simulink model "assm1023"  (R2017a)
settings: Solver=VariableStepAuto  StartTime=0.0  StopTime=inf  RelTol=1e-3
libraries: mblibv1 x33, simulink x5
settings Model: Creator=phoenix  LastModifiedBy=phoenix
settings SimMechanicsCC: VisOnUpdateDiagram=on  VisDuringSimulation=on

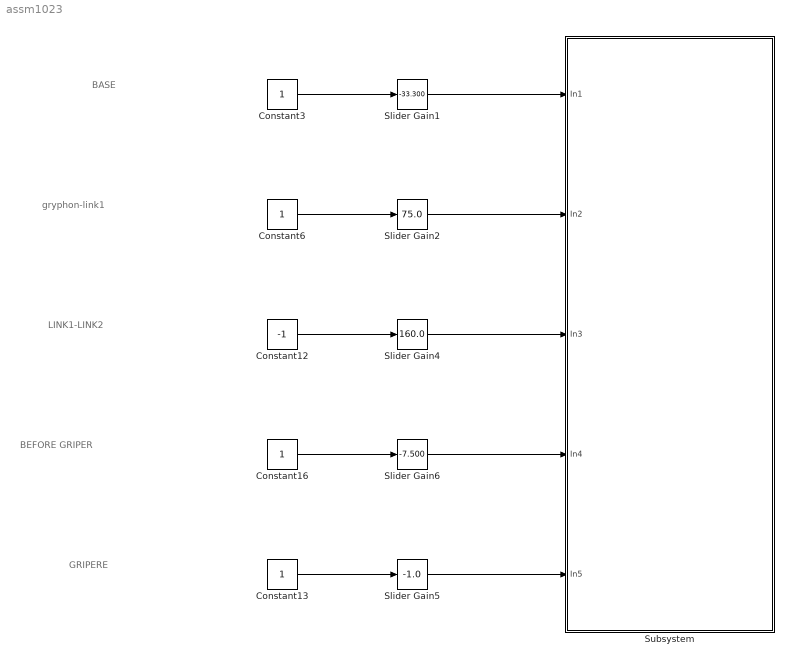
== system assm1023 ==
  note: BASE
  note: gryphon-link1
  note: LINK1-LINK2
  note: BEFORE GRIPER
  note: GRIPERE
  Constant12 : Constant  Value=-1
  Constant{3,6,13,16} (4 alike) : Constant
  Slider Gain1 : simulink/Math Operations/Slider Gain  gain=-33.300  low=-35  high=135
  Slider Gain2 : simulink/Math Operations/Slider Gain  gain=75.0  low=-15  high=75
  Slider Gain4 : simulink/Math Operations/Slider Gain  gain=160.0  low=10  high=160
  Slider Gain5 : simulink/Math Operations/Slider Gain  gain=-1.0  low=-1  high=30
  Slider Gain6 : simulink/Math Operations/Slider Gain  gain=-7.500  low=-90  high=60
  Subsystem : Subsystem
  wires:
  Slider Gain1/1 -> Subsystem/1(In1)
  Constant3/1 -> Slider Gain1/1
  Constant6/1 -> Slider Gain2/1
  Slider Gain2/1 -> Subsystem/2(In2)
  Slider Gain4/1 -> Subsystem/3(In3)
  Constant12/1 -> Slider Gain4/1
  Slider Gain6/1 -> Subsystem/4(In4)
  Constant16/1 -> Slider Gain6/1
  Constant13/1 -> Slider Gain5/1
  Slider Gain5/1 -> Subsystem/5(In5)

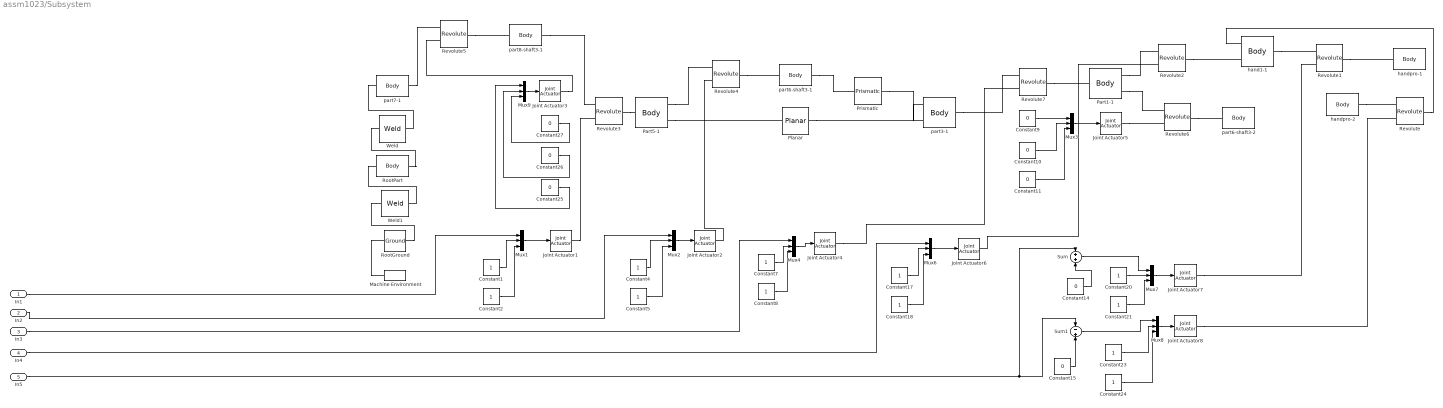
== system assm1023/Subsystem ==
  In1 : Inport
  In2 : Inport  Port=2
  In3 : Inport  Port=3
  In4 : Inport  Port=4
  In5 : Inport  Port=5
  Constant{1..2,4..5,7..8,17..18,20..21,23..24} (12 alike) : Constant
  Constant{9..11,14..15,25..27} (8 alike) : Constant  Value=0
  Joint Actuator{1..8} (8 alike) : mblibv1/Sensors &  Actuators/Joint Actuator  UpdateFromCAD=off  PhysicalDomain=Mechanical  PortType=blob  ActuationStyle=Motion  AngleUnits=deg  ArcVelocityUnits=deg/s  ArcAccelerationUnits=deg/s^2  CoordPositionUnits=m  VelocityUnits=m/s  AccelerationUnits=m/s^2  ForceUnits=N  TorqueUnits=N*m  ActiveIO=on  Width=3  DialogClass=MechanicalActuatorBlock  Primitive=R1  ReferenceFrame=Absolute (World)
      settings: SourceProductName=Simscape Multibody  SourceProductBaseCode=MS
  Machine Environment : mblibv1/Bodies/Machine Environment  PortType=env  PhysicalDomain=Mechanical  DialogTemplateClass=MECH.MachineEnvironment  SyncWhenCopied=off  Gravity=[0 -9.81 0]  GravityUnits=m/s^2  GravityAsSignal=off  Dimensionality=Auto-detect  AnalysisType=Forward dynamics  LinearAssemblyTolerance=1e-3  LinearAssemblyToleranceUnits=m  AngularAssemblyTolerance=1e-3  AngularAssemblyToleranceUnits=rad  ConstraintSolverType=Stabilizing  ConstraintRelTolerance=1e-4  ConstraintAbsTolerance=1e-4  UseRobustSingularityHandling=off  RedundancyAnalysisToleranceType=Automatically select tolerance  RedundancyAnalysisTolerance=1e-14  StatePerturbationType=Fixed  PerturbationSize=1e-5  VisualizeMachine=on  BodyVisualizationType=Use model default body geometries  BodyColorSelMode=Use model default  DefaultBodyColor=[1 0 0]
      settings: SourceProductName=Simscape Multibody  SourceProductBaseCode=MS
  Mux{1..4,6..9} (8 alike) : Mux  Inputs=3
  Part1-1 : mblibv1/Bodies/Body  LConnTagsString=CS4  RConnTagsString=CS2|CS3  UpdateFromCAD=on  DialogClass=MechanicalBodyBlock  Mass=9.49978  MassUnits=kg  InertiaUnits=kg*m^2  Inertia=[0.0164097,2.42302e-12,1.5644e-05;2.42302e-12,0.122916,-3.79927e-12;1.5644e-05,-3.79927e-12,0.124698]  Shape=Cylinder  ShapeDims=[1 1]  ShapeUnits=m  ShapeUse=false  Density=1  DensityUnits=kg/m^3  DensityUse=false  GraphicsMode=GFXFILE  GraphicsFileName=assm1023 - Part1-1.STL  BodyColorSelMode=COLORPALETTE  BodyColor=[0.898039;0.917647;0.929412]  AttachedToCS=CS1  CG=Right$CG$[0.0475798 0.46012 0.475956]$WORLD$WORLD$m$[-0.150782 -0.954807 -0.256141;0.861772 0 -0.507296;0.484369 -0.297226 0.822826]$3x3 Transform$rad$WORLD$false$none  WorkingFrames=Right$CS1$[0.122411 0.313454 0.408837]$WORLD$WORLD$m$[-0.150782 -0.954807 -0.256141;0.861772 0 -0.507296;0.484369 -0.297226 0.822826]$3x3 Transform$rad$WORLD$false$none#Right$CS2$[0.0598411 0.646508 0.594696]$WORLD$WORLD$m$[1 0 0;0 1 0;0 0 1]$3x3 Transform$rad$WORLD$true$none#Right$CS3$[0.00144863 0.44272 0.450878]$WORLD$WORLD$m$[1 0 0;0 1 0;0 0 1]$3x3 Transform$rad$WORLD$true$none#Left$CS4$[0.102331 0.44272 0.482283]$WORLD$WORLD$m$[1 0 0;0 1 0;0 0 1]$3x3 Transform$rad$WORLD$true$none  CGPos=[0.0475798 0.46012 0.475956]  CGRot=[-0.150782 -0.954807 -0.256141;0.861772 0 -0.507296;0.484369 -0.297226 0.822826]  CS0Pos=[]  CS0Rot=[]  CS1Pos=[0.122411 0.313454 0.408837]  CS1Rot=[-0.150782 -0.954807 -0.256141;0.861772 0 -0.507296;0.484369 -0.297226 0.822826]  CS2Pos=[0.0598411 0.646508 0.594696]  CS2Rot=[1 0 0;0 1 0;0 0 1]  CS3Pos=[0.00144863 0.44272 0.450878]  CS3Rot=[1 0 0;0 1 0;0 0 1]  CS4Pos=[0.102331 0.44272 0.482283]  CS4Rot=[1 0 0;0 1 0;0 0 1]  CS5Pos=[]  CS5Rot=[]  CS6Pos=[]  CS6Rot=[]  CS7Pos=[]  CS7Rot=[]  CS8Pos=[]  CS8Rot=[]  CS9Pos=[]  CS9Rot=[]  CS10Pos=[]  CS10Rot=[]  CS11Pos=[]  CS11Rot=[]  CS12Pos=[]  CS12Rot=[]  CS13Pos=[]  CS13Rot=[]  CS14Pos=[]  CS14Rot=[]  CS15Pos=[]  CS15Rot=[]  CS16Pos=[]  CS16Rot=[]  CS17Pos=[]  CS17Rot=[]  CS18Pos=[]  CS18Rot=[]  CS19Pos=[]  CS19Rot=[]  CS20Pos=[]  CS20Rot=[]
      settings: SourceProductName=Simscape Multibody  SourceProductBaseCode=MS
  Part5-1 : mblibv1/Bodies/Body  LConnTagsString=CS2  RConnTagsString=CS3|CS4  UpdateFromCAD=on  DialogClass=MechanicalBodyBlock  Mass=12.9081  MassUnits=kg  InertiaUnits=kg*m^2  Inertia=[0.0502011,-0.00109709,-3.42245e-05;-0.00109709,0.0708723,7.44572e-05;-3.42245e-05,7.44572e-05,0.0778857]  Shape=Cylinder  ShapeDims=[1 1]  ShapeUnits=m  ShapeUse=false  Density=1  DensityUnits=kg/m^3  DensityUse=false  GraphicsMode=GFXFILE  GraphicsFileName=assm1023 - Part5-1.STL  BodyColorSelMode=COLORPALETTE  BodyColor=[0.898039;0.917647;0.929412]  AttachedToCS=CS1  CG=Right$CG$[0.125791 0.354759 0.162602]$WORLD$WORLD$m$[-0.297226 0 -0.954807;0 1 0;0.954807 0 -0.297226]$3x3 Transform$rad$WORLD$false$none  WorkingFrames=Right$CS1$[0.125942 0.27534 0.161983]$WORLD$WORLD$m$[-0.297226 0 -0.954807;0 1 0;0.954807 0 -0.297226]$3x3 Transform$rad$WORLD$false$none#Left$CS2$[0.116431 0.27634 0.192537]$WORLD$WORLD$m$[1 0 0;0 1 0;0 0 1]$3x3 Transform$rad$WORLD$true$none#Right$CS3$[0.0325634 0.45934 0.226441]$WORLD$WORLD$m$[1 0 0;0 1 0;0 0 1]$3x3 Transform$rad$WORLD$true$none#Right$CS4$[0.225176 0.41534 0.0787147]$WORLD$WORLD$m$[1 0 0;0 1 0;0 0 1]$3x3 Transform$rad$WORLD$true$none  CGPos=[0.125791 0.354759 0.162602]  CGRot=[-0.297226 0 -0.954807;0 1 0;0.954807 0 -0.297226]  CS0Pos=[]  CS0Rot=[]  CS1Pos=[0.125942 0.27534 0.161983]  CS1Rot=[-0.297226 0 -0.954807;0 1 0;0.954807 0 -0.297226]  CS2Pos=[0.116431 0.27634 0.192537]  CS2Rot=[1 0 0;0 1 0;0 0 1]  CS3Pos=[0.0325634 0.45934 0.226441]  CS3Rot=[1 0 0;0 1 0;0 0 1]  CS4Pos=[0.225176 0.41534 0.0787147]  CS4Rot=[1 0 0;0 1 0;0 0 1]  CS5Pos=[]  CS5Rot=[]  CS6Pos=[]  CS6Rot=[]  CS7Pos=[]  CS7Rot=[]  CS8Pos=[]  CS8Rot=[]  CS9Pos=[]  CS9Rot=[]  CS10Pos=[]  CS10Rot=[]  CS11Pos=[]  CS11Rot=[]  CS12Pos=[]  CS12Rot=[]  CS13Pos=[]  CS13Rot=[]  CS14Pos=[]  CS14Rot=[]  CS15Pos=[]  CS15Rot=[]  CS16Pos=[]  CS16Rot=[]  CS17Pos=[]  CS17Rot=[]  CS18Pos=[]  CS18Rot=[]  CS19Pos=[]  CS19Rot=[]  CS20Pos=[]  CS20Rot=[]
      settings: SourceProductName=Simscape Multibody  SourceProductBaseCode=MS
  Planar : mblibv1/Joints/Planar  LConnTagsString=__newl0  RConnTagsString=__newr0  UpdateFromCAD=on  NumSAPorts=0  CutJoint=off  MarkAsCut=off  Primitives=prismatic_prismatic  PrimitiveProps=P1$WORLD$[-0.214972,0.690575,0.690575]$prismatic#P2$WORLD$[0.205257,0.723261,-0.659366]$prismatic#R1$WORLD$[0.954807,0,0.297226]$revolute  DialogClass=JointBlock  P1Axis=[-0.214972,0.690575,0.690575]  P2Axis=[0.205257,0.723261,-0.659366]  R1Axis=[0.954807,0,0.297226]
      settings: SourceProductName=Simscape Multibody  SourceProductBaseCode=MS
  Prismatic : mblibv1/Joints/Prismatic  LConnTagsString=__newl0  RConnTagsString=__newr0  UpdateFromCAD=on  NumSAPorts=0  CutJoint=off  MarkAsCut=off  Primitives=prismatic  PrimitiveProps=P1$WORLD$[-0.954807,0,-0.297226]$prismatic  DialogClass=JointBlock  P1Axis=[-0.954807,0,-0.297226]
      settings: SourceProductName=Simscape Multibody  SourceProductBaseCode=MS
  Revolute : mblibv1/Joints/Revolute  LConnTagsString=__newl0|SA1  RConnTagsString=__newr0  UpdateFromCAD=on  NumSAPorts=1  CutJoint=off  MarkAsCut=off  Primitives=prismatic  PrimitiveProps=R1$World$[-0.25737,-0.500207,0.826773]$revolute  DialogClass=JointBlock  R1Axis=[-0.25737,-0.500207,0.826773]
      settings: SourceProductName=Simscape Multibody  SourceProductBaseCode=MS
  Revolute1 : mblibv1/Joints/Revolute  LConnTagsString=__newl0|SA1  RConnTagsString=__newr0  UpdateFromCAD=on  NumSAPorts=1  CutJoint=off  MarkAsCut=off  Primitives=prismatic  PrimitiveProps=R1$World$[0.25737,0.500207,-0.826773]$revolute  DialogClass=JointBlock  R1Axis=[0.25737,0.500207,-0.826773]
      settings: SourceProductName=Simscape Multibody  SourceProductBaseCode=MS
  Revolute2 : mblibv1/Joints/Revolute  LConnTagsString=__newl0|SA1  RConnTagsString=__newr0  UpdateFromCAD=on  NumSAPorts=1  CutJoint=off  MarkAsCut=off  Primitives=prismatic  PrimitiveProps=R1$World$[-0.954807,0,-0.297226]$revolute  DialogClass=JointBlock  R1Axis=[-0.954807,0,-0.297226]
      settings: SourceProductName=Simscape Multibody  SourceProductBaseCode=MS
  Revolute3 : mblibv1/Joints/Revolute  LConnTagsString=__newl0|SA1  RConnTagsString=__newr0  UpdateFromCAD=on  NumSAPorts=1  CutJoint=off  MarkAsCut=off  Primitives=prismatic  PrimitiveProps=R1$World$[0,1,0]$revolute  DialogClass=JointBlock  R1Axis=[0,1,0]
      settings: SourceProductName=Simscape Multibody  SourceProductBaseCode=MS
  Revolute4 : mblibv1/Joints/Revolute  LConnTagsString=__newl0|SA1  RConnTagsString=__newr0  UpdateFromCAD=on  NumSAPorts=1  CutJoint=off  MarkAsCut=off  Primitives=prismatic  PrimitiveProps=R1$World$[-0.954807,0,-0.297226]$revolute  DialogClass=JointBlock  R1Axis=[-0.954807,0,-0.297226]
      settings: SourceProductName=Simscape Multibody  SourceProductBaseCode=MS
  Revolute5 : mblibv1/Joints/Revolute  LConnTagsString=__newl0|SA1  RConnTagsString=__newr0  UpdateFromCAD=on  NumSAPorts=1  CutJoint=off  MarkAsCut=off  Primitives=prismatic  PrimitiveProps=R1$World$[0,1,0]$revolute  DialogClass=JointBlock  R1Axis=[0,1,0]
      settings: SourceProductName=Simscape Multibody  SourceProductBaseCode=MS
  Revolute6 : mblibv1/Joints/Revolute  LConnTagsString=__newl0|SA1  RConnTagsString=__newr0  UpdateFromCAD=on  NumSAPorts=1  CutJoint=off  MarkAsCut=off  Primitives=prismatic  PrimitiveProps=R1$World$[0.954807,0,0.297226]$revolute  DialogClass=JointBlock  R1Axis=[0.954807,0,0.297226]
      settings: SourceProductName=Simscape Multibody  SourceProductBaseCode=MS
  Revolute7 : mblibv1/Joints/Revolute  LConnTagsString=__newl0|SA1  RConnTagsString=__newr0  UpdateFromCAD=on  NumSAPorts=1  CutJoint=off  MarkAsCut=off  Primitives=prismatic  PrimitiveProps=R1$World$[-0.954807,0,-0.297226]$revolute  DialogClass=JointBlock  R1Axis=[-0.954807,0,-0.297226]
      settings: SourceProductName=Simscape Multibody  SourceProductBaseCode=MS
  RootGround : mblibv1/Bodies/Ground  UpdateFromCAD=on  LeftPortType=env  RightPortType=workingframe  PhysicalDomain=Mechanical  DialogClass=GroundBlock  CoordPosition=[0.152895,0.40303,0.278658]  CoordPositionUnits=m  StateVectorMgrId=3  MachineId=[3 0]  ShowEnvPort=on  ParameterChecksum=[3598566596, 1641925801, 2828707792, 2140810860]  TopologyChecksum=[3969505370, 1508083990, 4183720490, 1127599918]
      settings: SourceProductName=Simscape Multibody  SourceProductBaseCode=MS
  RootPart : mblibv1/Bodies/Body  LConnTagsString=CS3  RConnTagsString=CS2  UpdateFromCAD=on  DialogClass=MechanicalBodyBlock  Mass=0  MassUnits=kg  InertiaUnits=kg*m^2  Inertia=[0,0,0;0,0,0;0,0,0]  Shape=Cylinder  ShapeDims=[1 1]  ShapeUnits=m  ShapeUse=false  Density=1  DensityUnits=kg/m^3  DensityUse=false  GraphicsMode=MACHINE_DEFAULT  BodyColorSelMode=MACHINE_DEFAULT  BodyColor=[1;0;0]  AttachedToCS=CS1  CG=Right$CG$[0.152895 0.40303 0.278658]$WORLD$WORLD$m$[1 0 0;0 1 0;0 0 1]$3x3 Transform$rad$WORLD$false$none  WorkingFrames=Right$CS1$[0 0 0]$WORLD$WORLD$m$[1 0 0;0 1 0;0 0 1]$3x3 Transform$rad$WORLD$false$none#Right$CS2$[0.0693468 0.0985547 0.192537]$WORLD$WORLD$m$[1 0 0;0 1 0;0 0 1]$3x3 Transform$rad$WORLD$true$none#Left$CS3$[0.152895 0.40303 0.278658]$WORLD$WORLD$m$[1 0 0;0 1 0;0 0 1]$3x3 Transform$rad$WORLD$true$none  CGPos=[0.152895 0.40303 0.278658]  CGRot=[1 0 0;0 1 0;0 0 1]  CS0Pos=[]  CS0Rot=[]  CS1Pos=[0 0 0]  CS1Rot=[1 0 0;0 1 0;0 0 1]  CS2Pos=[0.0693468 0.0985547 0.192537]  CS2Rot=[1 0 0;0 1 0;0 0 1]  CS3Pos=[0.152895 0.40303 0.278658]  CS3Rot=[1 0 0;0 1 0;0 0 1]  CS4Pos=[]  CS4Rot=[]  CS5Pos=[]  CS5Rot=[]  CS6Pos=[]  CS6Rot=[]  CS7Pos=[]  CS7Rot=[]  CS8Pos=[]  CS8Rot=[]  CS9Pos=[]  CS9Rot=[]  CS10Pos=[]  CS10Rot=[]  CS11Pos=[]  CS11Rot=[]  CS12Pos=[]  CS12Rot=[]  CS13Pos=[]  CS13Rot=[]  CS14Pos=[]  CS14Rot=[]  CS15Pos=[]  CS15Rot=[]  CS16Pos=[]  CS16Rot=[]  CS17Pos=[]  CS17Rot=[]  CS18Pos=[]  CS18Rot=[]  CS19Pos=[]  CS19Rot=[]  CS20Pos=[]  CS20Rot=[]
      settings: SourceProductName=Simscape Multibody  SourceProductBaseCode=MS
  Sum : Sum  Inputs=2
  Sum1 : Sum  Inputs=-+
  Weld : mblibv1/Joints/Weld  LConnTagsString=__newl0  RConnTagsString=__newr0  UpdateFromCAD=on  NumSAPorts=0  CutJoint=off  MarkAsCut=off  Primitives=weld  PrimitiveProps=W$WORLD$[0.57735,0.57735,0.57735]$weld  DialogClass=JointBlock  WAxis=[0.57735,0.57735,0.57735]
      settings: SourceProductName=Simscape Multibody  SourceProductBaseCode=MS
  Weld1 : mblibv1/Joints/Weld  LConnTagsString=__newl0  RConnTagsString=__newr0  UpdateFromCAD=on  NumSAPorts=0  CutJoint=off  MarkAsCut=off  Primitives=weld  PrimitiveProps=W$WORLD$[0.57735,0.57735,0.57735]$weld  DialogClass=JointBlock  WAxis=[0.57735,0.57735,0.57735]
      settings: SourceProductName=Simscape Multibody  SourceProductBaseCode=MS
  hand1-1 : mblibv1/Bodies/Body  LConnTagsString=CS2|CS4  RConnTagsString=CS3  UpdateFromCAD=on  DialogClass=MechanicalBodyBlock  Mass=0.148858  MassUnits=kg  InertiaUnits=kg*m^2  Inertia=[5.84343e-05,0,6.12626e-11;0,5.25166e-05,-5.81462e-11;6.12626e-11,-5.81462e-11,0.000105157]  Shape=Cylinder  ShapeDims=[1 1]  ShapeUnits=m  ShapeUse=false  Density=1  DensityUnits=kg/m^3  DensityUse=false  GraphicsMode=GFXFILE  GraphicsFileName=assm1023 - hand1-1.STL  BodyColorSelMode=COLORPALETTE  BodyColor=[0.647059;0.619608;0.588235]  AttachedToCS=CS1  CG=Right$CG$[0.00991066 0.675946 0.596964]$WORLD$WORLD$m$[-0.148675 0.954807 0.25737;0.865906 0 0.500207;0.477601 0.297226 -0.826773]$3x3 Transform$rad$WORLD$false$none  WorkingFrames=Right$CS1$[-0.0394589 0.646508 0.563785]$WORLD$WORLD$m$[-0.148675 0.954807 0.25737;0.865906 0 0.500207;0.477601 0.297226 -0.826773]$3x3 Transform$rad$WORLD$false$none#Left$CS2$[0.0024947 0.695768 0.6006]$WORLD$WORLD$m$[1 0 0;0 1 0;0 0 1]$3x3 Transform$rad$WORLD$true$none#Right$CS3$[0.0139524 0.695768 0.604167]$WORLD$WORLD$m$[1 0 0;0 1 0;0 0 1]$3x3 Transform$rad$WORLD$true$none#Left$CS4$[0.0598411 0.646508 0.594696]$WORLD$WORLD$m$[1 0 0;0 1 0;0 0 1]$3x3 Transform$rad$WORLD$true$none  CGPos=[0.00991066 0.675946 0.596964]  CGRot=[-0.148675 0.954807 0.25737;0.865906 0 0.500207;0.477601 0.297226 -0.826773]  CS0Pos=[]  CS0Rot=[]  CS1Pos=[-0.0394589 0.646508 0.563785]  CS1Rot=[-0.148675 0.954807 0.25737;0.865906 0 0.500207;0.477601 0.297226 -0.826773]  CS2Pos=[0.0024947 0.695768 0.6006]  CS2Rot=[1 0 0;0 1 0;0 0 1]  CS3Pos=[0.0139524 0.695768 0.604167]  CS3Rot=[1 0 0;0 1 0;0 0 1]  CS4Pos=[0.0598411 0.646508 0.594696]  CS4Rot=[1 0 0;0 1 0;0 0 1]  CS5Pos=[]  CS5Rot=[]  CS6Pos=[]  CS6Rot=[]  CS7Pos=[]  CS7Rot=[]  CS8Pos=[]  CS8Rot=[]  CS9Pos=[]  CS9Rot=[]  CS10Pos=[]  CS10Rot=[]  CS11Pos=[]  CS11Rot=[]  CS12Pos=[]  CS12Rot=[]  CS13Pos=[]  CS13Rot=[]  CS14Pos=[]  CS14Rot=[]  CS15Pos=[]  CS15Rot=[]  CS16Pos=[]  CS16Rot=[]  CS17Pos=[]  CS17Rot=[]  CS18Pos=[]  CS18Rot=[]  CS19Pos=[]  CS19Rot=[]  CS20Pos=[]  CS20Rot=[]
      settings: SourceProductName=Simscape Multibody  SourceProductBaseCode=MS
  handpro-1 : mblibv1/Bodies/Body  LConnTagsString=CS2  UpdateFromCAD=on  DialogClass=MechanicalBodyBlock  Mass=0.0310979  MassUnits=kg  InertiaUnits=kg*m^2  Inertia=[1.92545e-05,2.95676e-10,-1.69822e-06;2.95676e-10,2.09172e-05,-6.71129e-10;-1.69822e-06,-6.71129e-10,1.86479e-06]  Shape=Cylinder  ShapeDims=[1 1]  ShapeUnits=m  ShapeUse=false  Density=1  DensityUnits=kg/m^3  DensityUse=false  GraphicsMode=GFXFILE  GraphicsFileName=assm1023 - handpro-1.STL  BodyColorSelMode=COLORPALETTE  BodyColor=[0.647059;0.619608;0.588235]  AttachedToCS=CS1  CG=Right$CG$[0.0157979 0.728863 0.630692]$WORLD$WORLD$m$[-0.956473 0.25737 0.137549;0.0100807 0.500207 -0.865847;-0.291646 -0.826773 -0.481029]$3x3 Transform$rad$WORLD$false$none  WorkingFrames=Right$CS1$[0.00569132 0.690926 0.610519]$WORLD$WORLD$m$[-0.956473 0.25737 0.137549;0.0100807 0.500207 -0.865847;-0.291646 -0.826773 -0.481029]$3x3 Transform$rad$WORLD$false$none#Left$CS2$[0.0139524 0.695768 0.604167]$WORLD$WORLD$m$[1 0 0;0 1 0;0 0 1]$3x3 Transform$rad$WORLD$true$none  CGPos=[0.0157979 0.728863 0.630692]  CGRot=[-0.956473 0.25737 0.137549;0.0100807 0.500207 -0.865847;-0.291646 -0.826773 -0.481029]  CS0Pos=[]  CS0Rot=[]  CS1Pos=[0.00569132 0.690926 0.610519]  CS1Rot=[-0.956473 0.25737 0.137549;0.0100807 0.500207 -0.865847;-0.291646 -0.826773 -0.481029]  CS2Pos=[0.0139524 0.695768 0.604167]  CS2Rot=[1 0 0;0 1 0;0 0 1]  CS3Pos=[]  CS3Rot=[]  CS4Pos=[]  CS4Rot=[]  CS5Pos=[]  CS5Rot=[]  CS6Pos=[]  CS6Rot=[]  CS7Pos=[]  CS7Rot=[]  CS8Pos=[]  CS8Rot=[]  CS9Pos=[]  CS9Rot=[]  CS10Pos=[]  CS10Rot=[]  CS11Pos=[]  CS11Rot=[]  CS12Pos=[]  CS12Rot=[]  CS13Pos=[]  CS13Rot=[]  CS14Pos=[]  CS14Rot=[]  CS15Pos=[]  CS15Rot=[]  CS16Pos=[]  CS16Rot=[]  CS17Pos=[]  CS17Rot=[]  CS18Pos=[]  CS18Rot=[]  CS19Pos=[]  CS19Rot=[]  CS20Pos=[]  CS20Rot=[]
      settings: SourceProductName=Simscape Multibody  SourceProductBaseCode=MS
  handpro-2 : mblibv1/Bodies/Body  RConnTagsString=CS2  UpdateFromCAD=on  DialogClass=MechanicalBodyBlock  Mass=0.0310979  MassUnits=kg  InertiaUnits=kg*m^2  Inertia=[1.92545e-05,2.95676e-10,-1.69822e-06;2.95676e-10,2.09172e-05,-6.71129e-10;-1.69822e-06,-6.71129e-10,1.86479e-06]  Shape=Cylinder  ShapeDims=[1 1]  ShapeUnits=m  ShapeUse=false  Density=1  DensityUnits=kg/m^3  DensityUse=false  GraphicsMode=GFXFILE  GraphicsFileName=assm1023 - handpro-2.STL  BodyColorSelMode=COLORPALETTE  BodyColor=[0.647059;0.619608;0.588235]  AttachedToCS=CS1  CG=Right$CG$[-0.014809 0.728695 0.621061]$WORLD$WORLD$m$[0.949734 -0.25737 0.178231;0.0268696 -0.500207 -0.865489;0.311903 0.826773 -0.468148]$3x3 Transform$rad$WORLD$false$none  WorkingFrames=Right$CS1$[0.0081931 0.695929 0.602471]$WORLD$WORLD$m$[0.949734 -0.25737 0.178231;0.0268696 -0.500207 -0.865489;0.311903 0.826773 -0.468148]$3x3 Transform$rad$WORLD$false$none#Right$CS2$[0.0024947 0.695768 0.6006]$WORLD$WORLD$m$[1 0 0;0 1 0;0 0 1]$3x3 Transform$rad$WORLD$true$none  CGPos=[-0.014809 0.728695 0.621061]  CGRot=[0.949734 -0.25737 0.178231;0.0268696 -0.500207 -0.865489;0.311903 0.826773 -0.468148]  CS0Pos=[]  CS0Rot=[]  CS1Pos=[0.0081931 0.695929 0.602471]  CS1Rot=[0.949734 -0.25737 0.178231;0.0268696 -0.500207 -0.865489;0.311903 0.826773 -0.468148]  CS2Pos=[0.0024947 0.695768 0.6006]  CS2Rot=[1 0 0;0 1 0;0 0 1]  CS3Pos=[]  CS3Rot=[]  CS4Pos=[]  CS4Rot=[]  CS5Pos=[]  CS5Rot=[]  CS6Pos=[]  CS6Rot=[]  CS7Pos=[]  CS7Rot=[]  CS8Pos=[]  CS8Rot=[]  CS9Pos=[]  CS9Rot=[]  CS10Pos=[]  CS10Rot=[]  CS11Pos=[]  CS11Rot=[]  CS12Pos=[]  CS12Rot=[]  CS13Pos=[]  CS13Rot=[]  CS14Pos=[]  CS14Rot=[]  CS15Pos=[]  CS15Rot=[]  CS16Pos=[]  CS16Rot=[]  CS17Pos=[]  CS17Rot=[]  CS18Pos=[]  CS18Rot=[]  CS19Pos=[]  CS19Rot=[]  CS20Pos=[]  CS20Rot=[]
      settings: SourceProductName=Simscape Multibody  SourceProductBaseCode=MS
  part3-1 : mblibv1/Bodies/Body  LConnTagsString=CS2|CS3  RConnTagsString=CS4  UpdateFromCAD=on  DialogClass=MechanicalBodyBlock  Mass=22.0701  MassUnits=kg  InertiaUnits=kg*m^2  Inertia=[0.0642769,-0.00328587,0.00032545;-0.00328587,0.520617,9.03636e-05;0.00032545,9.03636e-05,0.499968]  Shape=Cylinder  ShapeDims=[1 1]  ShapeUnits=m  ShapeUse=false  Density=1  DensityUnits=kg/m^3  DensityUse=false  GraphicsMode=GFXFILE  GraphicsFileName=assm1023 - part3-1.STL  BodyColorSelMode=COLORPALETTE  BodyColor=[0.898039;0.917647;0.929412]  AttachedToCS=CS1  CG=Right$CG$[0.231238 0.460228 0.274716]$WORLD$WORLD$m$[-0.296408 0.954807 -0.022037;-0.0741422 0 0.997248;0.952179 0.297226 0.0707915]$3x3 Transform$rad$WORLD$false$none  WorkingFrames=Right$CS1$[0.251369 0.478246 0.0282195]$WORLD$WORLD$m$[-0.296408 0.954807 -0.022037;-0.0741422 0 0.997248;0.952179 0.297226 0.0707915]$3x3 Transform$rad$WORLD$false$none#Left$CS2$[0.225176 0.41534 0.0787147]$WORLD$WORLD$m$[1 0 0;0 1 0;0 0 1]$3x3 Transform$rad$WORLD$true$none#Left$CS3$[0.175784 0.45934 0.271025]$WORLD$WORLD$m$[1 0 0;0 1 0;0 0 1]$3x3 Transform$rad$WORLD$true$none#Right$CS4$[0.102331 0.44272 0.482283]$WORLD$WORLD$m$[1 0 0;0 1 0;0 0 1]$3x3 Transform$rad$WORLD$true$none  CGPos=[0.231238 0.460228 0.274716]  CGRot=[-0.296408 0.954807 -0.022037;-0.0741422 0 0.997248;0.952179 0.297226 0.0707915]  CS0Pos=[]  CS0Rot=[]  CS1Pos=[0.251369 0.478246 0.0282195]  CS1Rot=[-0.296408 0.954807 -0.022037;-0.0741422 0 0.997248;0.952179 0.297226 0.0707915]  CS2Pos=[0.225176 0.41534 0.0787147]  CS2Rot=[1 0 0;0 1 0;0 0 1]  CS3Pos=[0.175784 0.45934 0.271025]  CS3Rot=[1 0 0;0 1 0;0 0 1]  CS4Pos=[0.102331 0.44272 0.482283]  CS4Rot=[1 0 0;0 1 0;0 0 1]  CS5Pos=[]  CS5Rot=[]  CS6Pos=[]  CS6Rot=[]  CS7Pos=[]  CS7Rot=[]  CS8Pos=[]  CS8Rot=[]  CS9Pos=[]  CS9Rot=[]  CS10Pos=[]  CS10Rot=[]  CS11Pos=[]  CS11Rot=[]  CS12Pos=[]  CS12Rot=[]  CS13Pos=[]  CS13Rot=[]  CS14Pos=[]  CS14Rot=[]  CS15Pos=[]  CS15Rot=[]  CS16Pos=[]  CS16Rot=[]  CS17Pos=[]  CS17Rot=[]  CS18Pos=[]  CS18Rot=[]  CS19Pos=[]  CS19Rot=[]  CS20Pos=[]  CS20Rot=[]
      settings: SourceProductName=Simscape Multibody  SourceProductBaseCode=MS
  part6-shaft3-1 : mblibv1/Bodies/Body  LConnTagsString=CS2  RConnTagsString=CS3  UpdateFromCAD=on  DialogClass=MechanicalBodyBlock  Mass=0.648047  MassUnits=kg  InertiaUnits=kg*m^2  Inertia=[0.00229722,6.91896e-13,5.79579e-13;6.91896e-13,0.000112055,8.6782e-12;5.79579e-13,8.6782e-12,0.00229726]  Shape=Cylinder  ShapeDims=[1 1]  ShapeUnits=m  ShapeUse=false  Density=1  DensityUnits=kg/m^3  DensityUse=false  GraphicsMode=GFXFILE  GraphicsFileName=assm1023 - part6-shaft3-1.STL  BodyColorSelMode=COLORPALETTE  BodyColor=[0.647059;0.619608;0.588235]  AttachedToCS=CS1  CG=Right$CG$[0.115944 0.45934 0.252397]$WORLD$WORLD$m$[0.0145945 -0.954807 0.296868;-0.998794 0 0.0491024;-0.0468833 -0.297226 -0.953655]$3x3 Transform$rad$WORLD$false$none  WorkingFrames=Right$CS1$[0.213977 0.45934 0.282914]$WORLD$WORLD$m$[0.0145945 -0.954807 0.296868;-0.998794 0 0.0491024;-0.0468833 -0.297226 -0.953655]$3x3 Transform$rad$WORLD$false$none#Left$CS2$[0.0325634 0.45934 0.226441]$WORLD$WORLD$m$[1 0 0;0 1 0;0 0 1]$3x3 Transform$rad$WORLD$true$none#Right$CS3$[0.213977 0.45934 0.282914]$WORLD$WORLD$m$[1 0 0;0 1 0;0 0 1]$3x3 Transform$rad$WORLD$true$none  CGPos=[0.115944 0.45934 0.252397]  CGRot=[0.0145945 -0.954807 0.296868;-0.998794 0 0.0491024;-0.0468833 -0.297226 -0.953655]  CS0Pos=[]  CS0Rot=[]  CS1Pos=[0.213977 0.45934 0.282914]  CS1Rot=[0.0145945 -0.954807 0.296868;-0.998794 0 0.0491024;-0.0468833 -0.297226 -0.953655]  CS2Pos=[0.0325634 0.45934 0.226441]  CS2Rot=[1 0 0;0 1 0;0 0 1]  CS3Pos=[0.213977 0.45934 0.282914]  CS3Rot=[1 0 0;0 1 0;0 0 1]  CS4Pos=[]  CS4Rot=[]  CS5Pos=[]  CS5Rot=[]  CS6Pos=[]  CS6Rot=[]  CS7Pos=[]  CS7Rot=[]  CS8Pos=[]  CS8Rot=[]  CS9Pos=[]  CS9Rot=[]  CS10Pos=[]  CS10Rot=[]  CS11Pos=[]  CS11Rot=[]  CS12Pos=[]  CS12Rot=[]  CS13Pos=[]  CS13Rot=[]  CS14Pos=[]  CS14Rot=[]  CS15Pos=[]  CS15Rot=[]  CS16Pos=[]  CS16Rot=[]  CS17Pos=[]  CS17Rot=[]  CS18Pos=[]  CS18Rot=[]  CS19Pos=[]  CS19Rot=[]  CS20Pos=[]  CS20Rot=[]
      settings: SourceProductName=Simscape Multibody  SourceProductBaseCode=MS
  part6-shaft3-2 : mblibv1/Bodies/Body  LConnTagsString=CS2  UpdateFromCAD=on  DialogClass=MechanicalBodyBlock  Mass=0.648047  MassUnits=kg  InertiaUnits=kg*m^2  Inertia=[0.00229722,6.91896e-13,5.79579e-13;6.91896e-13,0.000112055,8.6782e-12;5.79579e-13,8.6782e-12,0.00229726]  Shape=Cylinder  ShapeDims=[1 1]  ShapeUnits=m  ShapeUse=false  Density=1  DensityUnits=kg/m^3  DensityUse=false  GraphicsMode=GFXFILE  GraphicsFileName=assm1023 - part6-shaft3-2.STL  BodyColorSelMode=COLORPALETTE  BodyColor=[0.647059;0.619608;0.588235]  AttachedToCS=CS1  CG=Right$CG$[0.0848294 0.44272 0.476834]$WORLD$WORLD$m$[0.0636487 -0.954807 -0.290331;0.976802 0 0.214142;-0.204465 -0.297226 0.932658]$3x3 Transform$rad$WORLD$false$none  WorkingFrames=Right$CS1$[0.182862 0.44272 0.507351]$WORLD$WORLD$m$[0.0636487 -0.954807 -0.290331;0.976802 0 0.214142;-0.204465 -0.297226 0.932658]$3x3 Transform$rad$WORLD$false$none#Left$CS2$[0.00144863 0.44272 0.450878]$WORLD$WORLD$m$[1 0 0;0 1 0;0 0 1]$3x3 Transform$rad$WORLD$true$none  CGPos=[0.0848294 0.44272 0.476834]  CGRot=[0.0636487 -0.954807 -0.290331;0.976802 0 0.214142;-0.204465 -0.297226 0.932658]  CS0Pos=[]  CS0Rot=[]  CS1Pos=[0.182862 0.44272 0.507351]  CS1Rot=[0.0636487 -0.954807 -0.290331;0.976802 0 0.214142;-0.204465 -0.297226 0.932658]  CS2Pos=[0.00144863 0.44272 0.450878]  CS2Rot=[1 0 0;0 1 0;0 0 1]  CS3Pos=[]  CS3Rot=[]  CS4Pos=[]  CS4Rot=[]  CS5Pos=[]  CS5Rot=[]  CS6Pos=[]  CS6Rot=[]  CS7Pos=[]  CS7Rot=[]  CS8Pos=[]  CS8Rot=[]  CS9Pos=[]  CS9Rot=[]  CS10Pos=[]  CS10Rot=[]  CS11Pos=[]  CS11Rot=[]  CS12Pos=[]  CS12Rot=[]  CS13Pos=[]  CS13Rot=[]  CS14Pos=[]  CS14Rot=[]  CS15Pos=[]  CS15Rot=[]  CS16Pos=[]  CS16Rot=[]  CS17Pos=[]  CS17Rot=[]  CS18Pos=[]  CS18Rot=[]  CS19Pos=[]  CS19Rot=[]  CS20Pos=[]  CS20Rot=[]
      settings: SourceProductName=Simscape Multibody  SourceProductBaseCode=MS
  part7-1 : mblibv1/Bodies/Body  LConnTagsString=CS2  RConnTagsString=CS3  UpdateFromCAD=on  DialogClass=MechanicalBodyBlock  Mass=1.72088  MassUnits=kg  InertiaUnits=kg*m^2  Inertia=[0.00316504,-0.000339953,0;-0.000339953,0.0102423,0;0,0,0.00747269]  Shape=Cylinder  ShapeDims=[1 1]  ShapeUnits=m  ShapeUse=false  Density=1  DensityUnits=kg/m^3  DensityUse=false  GraphicsMode=GFXFILE  GraphicsFileName=assm1023 - part7-1.STL  BodyColorSelMode=COLORPALETTE  BodyColor=[0.898039;0.917647;0.929412]  AttachedToCS=CS1  CG=Right$CG$[0.0693468 0.0985547 0.192537]$WORLD$WORLD$m$[1 0 0;0 1 0;0 0 1]$3x3 Transform$rad$WORLD$false$none  WorkingFrames=Right$CS1$[-0.058569 0.08734 0.270037]$WORLD$WORLD$m$[1 0 0;0 1 0;0 0 1]$3x3 Transform$rad$WORLD$false$none#Left$CS2$[0.0693468 0.0985547 0.192537]$WORLD$WORLD$m$[1 0 0;0 1 0;0 0 1]$3x3 Transform$rad$WORLD$true$none#Right$CS3$[0.116431 0.11134 0.192537]$WORLD$WORLD$m$[1 0 0;0 1 0;0 0 1]$3x3 Transform$rad$WORLD$true$none  CGPos=[0.0693468 0.0985547 0.192537]  CGRot=[1 0 0;0 1 0;0 0 1]  CS0Pos=[]  CS0Rot=[]  CS1Pos=[-0.058569 0.08734 0.270037]  CS1Rot=[1 0 0;0 1 0;0 0 1]  CS2Pos=[0.0693468 0.0985547 0.192537]  CS2Rot=[1 0 0;0 1 0;0 0 1]  CS3Pos=[0.116431 0.11134 0.192537]  CS3Rot=[1 0 0;0 1 0;0 0 1]  CS4Pos=[]  CS4Rot=[]  CS5Pos=[]  CS5Rot=[]  CS6Pos=[]  CS6Rot=[]  CS7Pos=[]  CS7Rot=[]  CS8Pos=[]  CS8Rot=[]  CS9Pos=[]  CS9Rot=[]  CS10Pos=[]  CS10Rot=[]  CS11Pos=[]  CS11Rot=[]  CS12Pos=[]  CS12Rot=[]  CS13Pos=[]  CS13Rot=[]  CS14Pos=[]  CS14Rot=[]  CS15Pos=[]  CS15Rot=[]  CS16Pos=[]  CS16Rot=[]  CS17Pos=[]  CS17Rot=[]  CS18Pos=[]  CS18Rot=[]  CS19Pos=[]  CS19Rot=[]  CS20Pos=[]  CS20Rot=[]
      settings: SourceProductName=Simscape Multibody  SourceProductBaseCode=MS
  part8-shaft3-1 : mblibv1/Bodies/Body  LConnTagsString=CS3  RConnTagsString=CS2  UpdateFromCAD=on  DialogClass=MechanicalBodyBlock  Mass=3.73221  MassUnits=kg  InertiaUnits=kg*m^2  Inertia=[0.0093072,0,0;0,0.0016795,0;0,0,0.0093072]  Shape=Cylinder  ShapeDims=[1 1]  ShapeUnits=m  ShapeUse=false  Density=1  DensityUnits=kg/m^3  DensityUse=false  GraphicsMode=GFXFILE  GraphicsFileName=assm1023 - part8-shaft3-1.STL  BodyColorSelMode=COLORPALETTE  BodyColor=[0.647059;0.619608;0.588235]  AttachedToCS=CS1  CG=Right$CG$[0.116431 0.19384 0.192537]$WORLD$WORLD$m$[0.836085 0 0.5486;0 1 0;-0.5486 0 0.836085]$3x3 Transform$rad$WORLD$false$none  WorkingFrames=Right$CS1$[0.116431 0.11134 0.192537]$WORLD$WORLD$m$[0.836085 0 0.5486;0 1 0;-0.5486 0 0.836085]$3x3 Transform$rad$WORLD$false$none#Right$CS2$[0.116431 0.27634 0.192537]$WORLD$WORLD$m$[1 0 0;0 1 0;0 0 1]$3x3 Transform$rad$WORLD$true$none#Left$CS3$[0.116431 0.11134 0.192537]$WORLD$WORLD$m$[1 0 0;0 1 0;0 0 1]$3x3 Transform$rad$WORLD$true$none  CGPos=[0.116431 0.19384 0.192537]  CGRot=[0.836085 0 0.5486;0 1 0;-0.5486 0 0.836085]  CS0Pos=[]  CS0Rot=[]  CS1Pos=[0.116431 0.11134 0.192537]  CS1Rot=[0.836085 0 0.5486;0 1 0;-0.5486 0 0.836085]  CS2Pos=[0.116431 0.27634 0.192537]  CS2Rot=[1 0 0;0 1 0;0 0 1]  CS3Pos=[0.116431 0.11134 0.192537]  CS3Rot=[1 0 0;0 1 0;0 0 1]  CS4Pos=[]  CS4Rot=[]  CS5Pos=[]  CS5Rot=[]  CS6Pos=[]  CS6Rot=[]  CS7Pos=[]  CS7Rot=[]  CS8Pos=[]  CS8Rot=[]  CS9Pos=[]  CS9Rot=[]  CS10Pos=[]  CS10Rot=[]  CS11Pos=[]  CS11Rot=[]  CS12Pos=[]  CS12Rot=[]  CS13Pos=[]  CS13Rot=[]  CS14Pos=[]  CS14Rot=[]  CS15Pos=[]  CS15Rot=[]  CS16Pos=[]  CS16Rot=[]  CS17Pos=[]  CS17Rot=[]  CS18Pos=[]  CS18Rot=[]  CS19Pos=[]  CS19Rot=[]  CS20Pos=[]  CS20Rot=[]
      settings: SourceProductName=Simscape Multibody  SourceProductBaseCode=MS
  wires:
  Constant24/1 -> Mux8/3
  Constant20/1 -> Mux7/2
  Mux7/1 -> Joint Actuator7/1
  Constant18/1 -> Mux6/3
  Mux9/1 -> Joint Actuator3/1
  Constant8/1 -> Mux4/3
  Constant7/1 -> Mux4/2
  Constant4/1 -> Mux2/2
  Mux2/1 -> Joint Actuator2/1
  Constant1/1 -> Mux1/2
  Mux4/1 -> Joint Actuator4/1
  Constant2/1 -> Mux1/3
  Mux1/1 -> Joint Actuator1/1
  Sum1/1 -> Mux8/1
  Constant17/1 -> Mux6/2
  Constant26/1 -> Mux9/2
  Constant27/1 -> Mux9/3
  Mux3/1 -> Joint Actuator5/1
  Constant10/1 -> Mux3/2
  Constant23/1 -> Mux8/2
  Constant11/1 -> Mux3/3
  Constant25/1 -> Mux9/1
  Constant21/1 -> Mux7/3
  Constant14/1 -> Sum/2
  Sum/1 -> Mux7/1
  Mux8/1 -> Joint Actuator8/1
  Constant5/1 -> Mux2/3
  Constant15/1 -> Sum1/2
  Constant9/1 -> Mux3/1
  Mux6/1 -> Joint Actuator6/1
  In1/1 -> Mux1/1
  In2/1 -> Mux2/1
  In3/1 -> Mux4/1
  In4/1 -> Mux6/1
  In5/1 -> Sum1/1, Sum/1
  connections:
  part6-shaft3-1/RConn1 -- Prismatic/LConn1
  Joint Actuator5/RConn1 -- Revolute6/LConn2
  Joint Actuator1/RConn1 -- Revolute3/LConn2
  Revolute7/RConn1 -- Part1-1/LConn1
  part3-1/RConn1 -- Revolute7/LConn1
  Joint Actuator3/RConn1 -- Revolute5/LConn2
  Joint Actuator6/RConn1 -- Revolute2/LConn2
  Prismatic/RConn1 -- part3-1/LConn2
  Revolute5/RConn1 -- part8-shaft3-1/LConn1
  RootGround/RConn1 -- Weld1/LConn1
  Joint Actuator7/RConn1 -- Revolute1/LConn2
  Joint Actuator8/RConn1 -- Revolute/LConn2
  part7-1/RConn1 -- Revolute5/LConn1
  Revolute6/RConn1 -- part6-shaft3-2/LConn1
  part8-shaft3-1/RConn1 -- Revolute3/LConn1
  Part1-1/RConn1 -- Revolute2/LConn1
  Revolute/RConn1 -- hand1-1/LConn1
  Revolute4/RConn1 -- part6-shaft3-1/LConn1
  Revolute3/RConn1 -- Part5-1/LConn1
  Part1-1/RConn2 -- Revolute6/LConn1
  Planar/RConn1 -- part3-1/LConn1
  Part5-1/RConn1 -- Revolute4/LConn1
  Joint Actuator2/RConn1 -- Revolute4/LConn2
  Revolute2/RConn1 -- hand1-1/LConn2
  Part5-1/RConn2 -- Planar/LConn1
  Weld1/RConn1 -- RootPart/LConn1
  RootPart/RConn1 -- Weld/LConn1
  Revolute1/RConn1 -- handpro-1/LConn1
  Joint Actuator4/RConn1 -- Revolute7/LConn2
  Weld/RConn1 -- part7-1/LConn1
  hand1-1/RConn1 -- Revolute1/LConn1
  RootGround/LConn1 -- Machine Environment/RConn1
  handpro-2/RConn1 -- Revolute/LConn1
